simulink model "Sistema4"  (R2026b)
settings: Solver=ode15s  StopTime=10  MaxStep=1E-2
libraries: slpidlib x1
settings Model: LastModifiedBy=Marcos Ancelmo
settings DataIOCC: DSMLogging=off  ReturnWorkspaceOutputs=off  SaveFormat=Array  SaveOutput=off  SignalLogging=off  TimeSaveName=t
settings DebuggingCC: AlgebraicLoopMsg=none  ArtificialAlgebraicLoopMsg=none  MaxConsecutiveZCsMsg=none

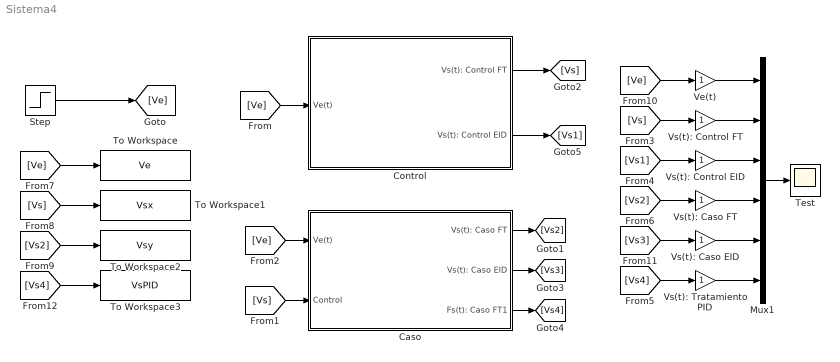
== system Sistema4 ==
  " Ve(t)" : Gain
  " Vs(t): Caso EID" : Gain
  " Vs(t): Caso FT" : Gain
  " Vs(t): Control EID" : Gain
  " Vs(t): Control FT" : Gain
  " Vs(t): Tratamiento PID" : Gain
  Caso : Subsystem
  Control : Subsystem
  Mux1 : Mux  Inputs=6
  Step : Step  Time=0  SampleTime=0
  Test : Scope
      settings: ActiveDisplayYMinimum=0.9900990042680653  ActiveDisplayYMaximum=0.99009901171000014
  To Workspace : ToWorkspace  VariableName=Ve  SampleTime=-1
  To Workspace1 : ToWorkspace  VariableName=Vsx  SampleTime=-1
  To Workspace2 : ToWorkspace  VariableName=Vsy  SampleTime=-1
  To Workspace3 : ToWorkspace  VariableName=VsPID  SampleTime=-1
  wires:
  [Ve] -> Control/1(Ve(t))
  Control/1(Vs(t): Control FT) -> [Vs]
  [Ve] -> Caso/1(Ve(t))
  Caso/1(Vs(t): Caso FT) -> [Vs2]
  Mux1/1 -> Test/1
  [Vs] -> " Vs(t): Control FT"/1
  [Vs1] -> " Vs(t): Control EID"/1
  Step/1 -> [Ve]
  Caso/2(Vs(t): Caso EID) -> [Vs3]
  [Vs2] -> " Vs(t): Caso FT"/1
  [Ve] -> " Ve(t)"/1
  " Vs(t): Control FT"/1 -> Mux1/2
  " Ve(t)"/1 -> Mux1/1
  " Vs(t): Control EID"/1 -> Mux1/3
  " Vs(t): Caso FT"/1 -> Mux1/4
  Control/2(Vs(t): Control EID) -> [Vs1]
  [Vs3] -> " Vs(t): Caso EID"/1
  " Vs(t): Caso EID"/1 -> Mux1/5
  [Vs] -> Caso/2(Control)
  Caso/3(Fs(t): Caso FT1) -> [Vs4]
  [Vs4] -> " Vs(t): Tratamiento PID"/1
  " Vs(t): Tratamiento PID"/1 -> Mux1/6
  [Ve] -> To Workspace/1
  [Vs] -> To Workspace1/1
  [Vs2] -> To Workspace2/1
  [Vs4] -> To Workspace3/1

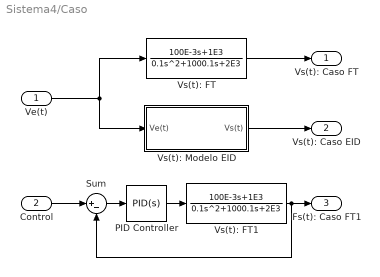
== system Sistema4/Caso ==
  Ve(t) : Inport
  Control : Inport  Port=2
  PID Controller : slpidlib/PID Controller  Controller=PID  Form=Parallel  TimeDomain=Continuous-time  UseExternalTs=off  SampleTime=-1  IntegratorMethod=Forward Euler  FilterMethod=Forward Euler  ControllerParametersSource=internal  P=13228.2789956596  I=32406234.0640177  UseKiTs=off  D=0.181178782186765  UseExternalDerivativeSource=off  N=50580.0841438419  UseFilter=on  TunerSelectOption=Transfer Function Based (PID Tuner App)  InitialConditionSource=internal  InitialConditionForIntegrator=0  InitialConditionForFilter=0  DifferentiatorICPrevScaledInput=0  ExternalReset=none  TrackingMode=off  Kt=1  LimitOutput=off  SatLimitsSource=internal  UpperSaturationLimit=inf  LowerSaturationLimit=-inf  LinearizeAsGain=on  AntiWindupMode=none  Kb=1  LimitIntegrator=off  UpperIntegratorSaturationLimit=inf  LowerIntegratorSaturationLimit=-inf  POutMin=[]  POutMax=[]  IOutMin=[]  IOutMax=[]  DOutMin=[]  DOutMax=[]  NOutMin=[]  NOutMax=[]  SumOutMin=[]  SumOutMax=[]  SaturationOutMin=[]  SaturationOutMax=[]  PParamMin=[]  PParamMax=[]  IParamMin=[]  IParamMax=[]  DParamMin=[]  DParamMax=[]  NParamMin=[]  NParamMax=[]  KbParamMin=[]  KbParamMax=[]  KtParamMin=[]  KtParamMax=[]  KbOutMin=[]  KbOutMax=[]  KtOutMin=[]  KtOutMax=[]  IntegratorOutMin=[]  IntegratorOutMax=[]  FilterOutMin=[]  FilterOutMax=[]  SumI1OutMin=[]  SumI1OutMax=[]  SumI2OutMin=[]  SumI2OutMax=[]  SumI3OutMin=[]  SumI3OutMax=[]  SumI4OutMin=[]  SumI4OutMax=[]  SumDOutMin=[]  SumDOutMax=[]  DifferentiatorOutMin=[]  DifferentiatorOutMax=[]  FilterDiffOutCoefMin=[]  FilterDiffOutCoefMax=[]  ReciprocalOutMin=[]  ReciprocalOutMax=[]  SumDenOutMin=[]  SumDenOutMax=[]  SumNumOutMin=[]  SumNumOutMax=[]  DivideOutMin=[]  DivideOutMax=[]  UdiffTsProdOutMin=[]  UdiffTsProdOutMax=[]  NTsProdOutMin=[]  NTsProdOutMax=[]  UintegralTsProdOutMin=[]  UintegralTsProdOutMax=[]  UngainTsProdOutMin=[]  UngainTsProdOutMax=[]  ClampingZeroOutDataTypeStr=Inherit: Inherit via back propagation  ClampingZeroOutMin=[]  ClampingZeroOutMax=[]  FilterDenConstantOutDataTypeStr=Inherit: Inherit via back propagation  FilterDenConstantOutMin=[]  FilterDenConstantOutMax=[]  PCopyOutDataTypeStr=Inherit: Inherit via back propagation  PCopyOutMin=[]  PCopyOutMax=[]  NCopyOutDataTypeStr=Inherit: Inherit via back propagation  NCopyOutMin=[]  NCopyOutMax=[]  IntegratorContinuousStateAttributes=''  IntegratorStateMustResolveToSignalObject=off  IntegratorRTWStateStorageClass=Auto  FilterContinuousStateAttributes=''  FilterStateMustResolveToSignalObject=off  FilterRTWStateStorageClass=Auto  ParallelPVariant=InternalParameters  IdealPVariant=Disabled  IVariant=InternalParameters  DVariant=InternalParameters  IntegratorVariant=Continuous  SatVariant=Disabled  AWVariant=Passthrough  PCopyVariant=Disabled  TRVariant=Disabled  FdbkBlocksVariant=Forward  IdealPFdbkVariant=Disabled  SatFdbkVariant=Disabled  DerivativeFilterVariant=ContFilter  NVariant=InternalParameters  NCopyVariant=Disabled  FilterICVariant=InternalICsFilter  IntegratorICVariant=InternalICs  ExternalResetVariant=Disabled  TRSumVariant=Passthrough  SumFdbkVariant=Disabled  SumVariant=Sum_PID  TsampFilterVariant=InternalTs  TsampNgainVariant=Passthrough  TsampIntegralVariant=Disabled_SignalSpec  ExternalSaturationOutDataTypeStr=Inherit: Same as second input  DerivativeSourceVariant=ErrorSignal  PreIntVariant=InternalPreInt
  Sum : Sum  Inputs=|+-
  Vs(t): FT : TransferFcn  Numerator=[100E-3, 1E3]  Denominator=[0.1, 1000.1, 2E3]
  Vs(t): FT1 : TransferFcn  Numerator=[100E-3, 1E3]  Denominator=[0.1, 1000.1, 2E3]
  Vs(t): Modelo EID : Subsystem
  Vs(t): Caso FT : Outport
  Vs(t): Caso EID : Outport  Port=2
  Fs(t): Caso FT1 : Outport  Port=3
  wires:
  Ve(t)/1 -> Vs(t): Modelo EID/1(Ve(t)), Vs(t): FT/1
  Vs(t): FT/1 -> Vs(t): Caso FT/1
  Vs(t): Modelo EID/1(Vs(t)) -> Vs(t): Caso EID/1
  Vs(t): FT1/1 -> Fs(t): Caso FT1/1, Sum/2
  Control/1 -> Sum/1
  PID Controller/1 -> Vs(t): FT1/1
  Sum/1 -> PID Controller/1

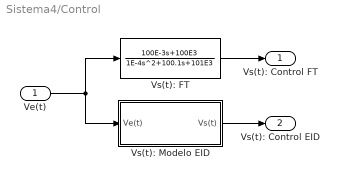
== system Sistema4/Control ==
  Ve(t) : Inport
  Vs(t): FT : TransferFcn  Numerator=[100E-3, 100E3]  Denominator=[1E-4, 100.1, 101E3]
  Vs(t): Modelo EID : Subsystem
  Vs(t): Control FT : Outport
  Vs(t): Control EID : Outport  Port=2
  wires:
  Ve(t)/1 -> Vs(t): Modelo EID/1(Ve(t)), Vs(t): FT/1
  Vs(t): FT/1 -> Vs(t): Control FT/1
  Vs(t): Modelo EID/1(Vs(t)) -> Vs(t): Control EID/1

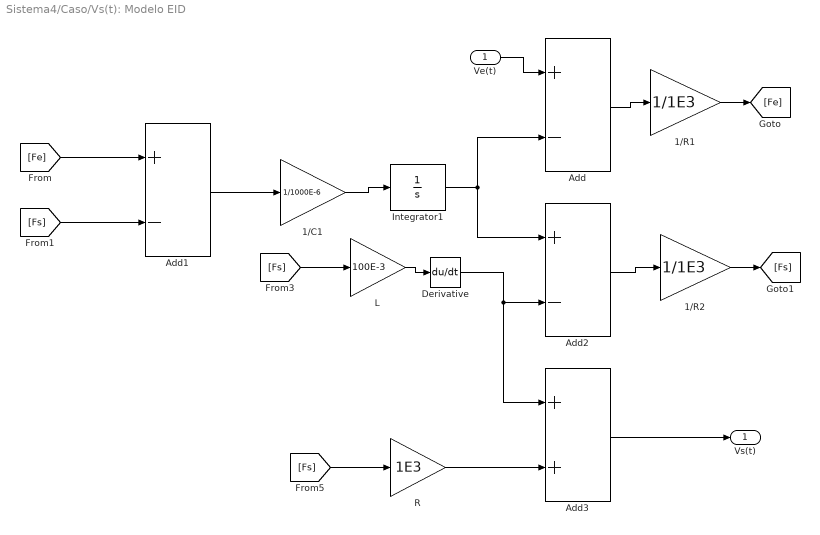
== system Sistema4/Caso/Vs(t): Modelo EID ==
  Ve(t) : Inport
  1/C1 : Gain  Gain=1/1000E-6
  1/R1 : Gain  Gain=1/1E3
  1/R2 : Gain  Gain=1/1E3
  Add : Sum  Inputs=+-
  Add1 : Sum  Inputs=+-
  Add2 : Sum  Inputs=+-
  Add3 : Sum
  Derivative : Derivative
  Integrator1 : Integrator
  L : Gain  Gain=100E-3
  R : Gain  Gain=1E3
  Vs(t) : Outport
  wires:
  1/R1/1 -> [Fe]
  [Fs] -> Add1/2
  [Fe] -> Add1/1
  [Fs] -> L/1
  Add/1 -> 1/R1/1
  [Fs] -> R/1
  1/C1/1 -> Integrator1/1
  Ve(t)/1 -> Add/1
  Add1/1 -> 1/C1/1
  Add2/1 -> 1/R2/1
  1/R2/1 -> [Fs]
  Add3/1 -> Vs(t)/1
  Integrator1/1 -> Add2/1, Add/2
  R/1 -> Add3/2
  L/1 -> Derivative/1
  Derivative/1 -> Add3/1, Add2/2

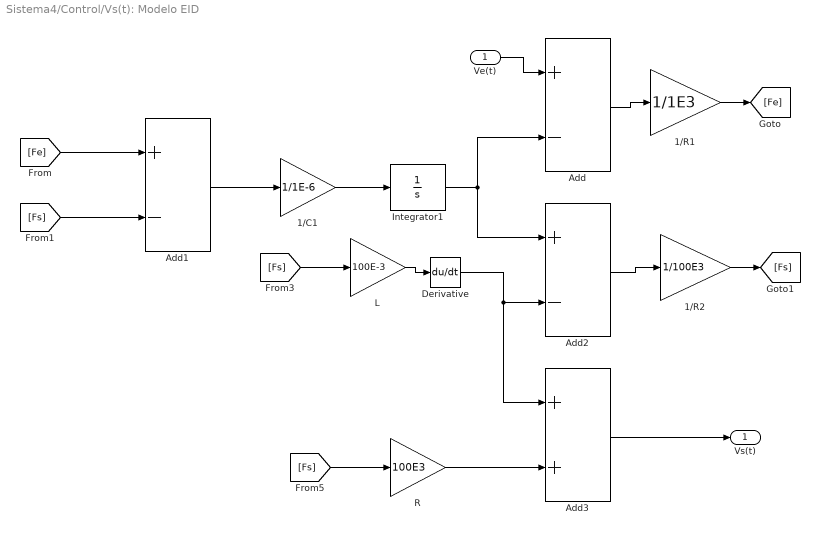
== system Sistema4/Control/Vs(t): Modelo EID ==
  Ve(t) : Inport
  1/C1 : Gain  Gain=1/1E-6
  1/R1 : Gain  Gain=1/1E3
  1/R2 : Gain  Gain=1/100E3
  Add : Sum  Inputs=+-
  Add1 : Sum  Inputs=+-
  Add2 : Sum  Inputs=+-
  Add3 : Sum
  Derivative : Derivative
  Integrator1 : Integrator
  L : Gain  Gain=100E-3
  R : Gain  Gain=100E3
  Vs(t) : Outport
  wires:
  1/R1/1 -> [Fe]
  [Fs] -> Add1/2
  [Fe] -> Add1/1
  [Fs] -> L/1
  Add/1 -> 1/R1/1
  [Fs] -> R/1
  1/C1/1 -> Integrator1/1
  Ve(t)/1 -> Add/1
  Add1/1 -> 1/C1/1
  Add2/1 -> 1/R2/1
  1/R2/1 -> [Fs]
  Add3/1 -> Vs(t)/1
  Integrator1/1 -> Add2/1, Add/2
  R/1 -> Add3/2
  L/1 -> Derivative/1
  Derivative/1 -> Add3/1, Add2/2
